simulink model "GP_DataCollection_2R"  (R2024a)
settings: Solver=ode4  StartTime=0.0  StopTime=6  FixedStep=0.001  RelTol=1e-3
model workspace (MAT data in the model file):
  p_hat.a1 = 1
  p_hat.a2 = 1
  p_hat.m1 = 2
  p_hat.m2 = 1
  p_hat.mm1 = 0.5
  p_hat.mm2 = 0.3
  p_hat.l1 = 0.5
  p_hat.l2 = 0.5
  p_hat.I1 = 0.166666666667
  p_hat.I2 = 0.0833333333333
  p_hat.kr1 = 50
  p_hat.kr2 = 50
  p_hat.Im1 = 0.0001
  p_hat.Im2 = 0.0001
  p_hat.g0 = 9.81
  p_real.a1 = 1
  p_real.a2 = 1
  p_real.m1 = 2
  p_real.m2 = 1
  p_real.mm1 = 0.5
  p_real.mm2 = 0.3
  p_real.l1 = 0.5
  p_real.l2 = 0.5
  p_real.I1 = 0.166666666667
  p_real.I2 = 0.0833333333333
  p_real.kr1 = 50
  p_real.kr2 = 50
  p_real.Im1 = 0.0001
  p_real.Im2 = 0.0001
  p_real.g0 = 9.81
undefined symbols (not defined in the file): dq0, Kd, Kp, q0
settings Model: Creator=Mariapaola  LastModifiedBy=Mariapaola

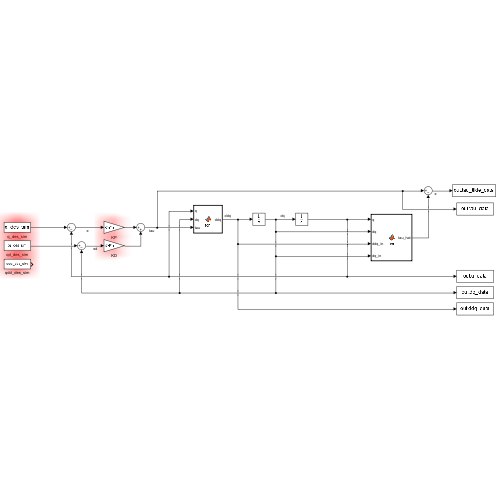
[thumbnail: Simulink's stored preview of the top-level diagram]
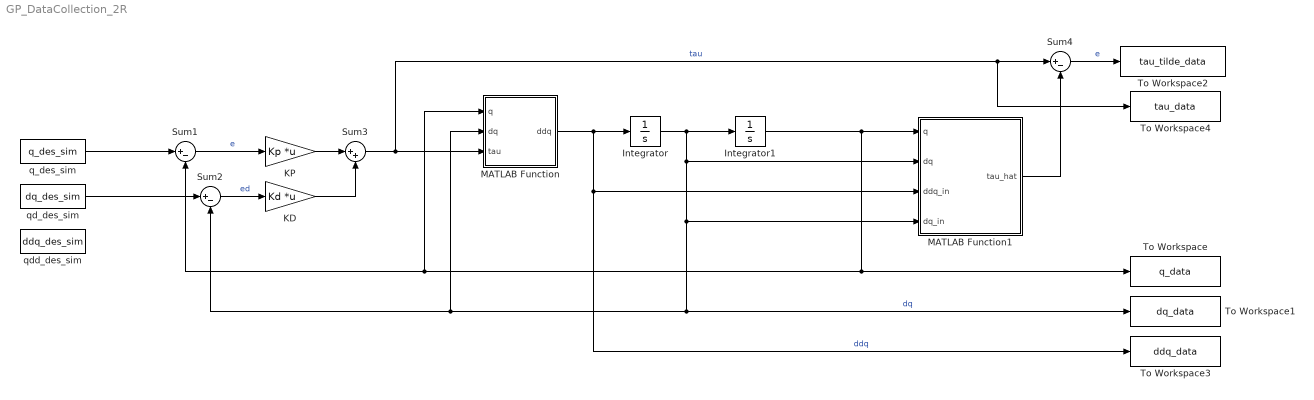
== system GP_DataCollection_2R ==
  Integrator : Integrator  InitialCondition=dq0
  Integrator1 : Integrator  InitialCondition=q0
  KD : Gain  Gain=Kd  Multiplication=Matrix(K*u)
  KP : Gain  Gain=Kp  Multiplication=Matrix(K*u)
  MATLAB Function : MATLAB Function  TreatAsAtomicUnit=on
  MATLAB Function1 : MATLAB Function  TreatAsAtomicUnit=on
  Sum1 : Sum  Inputs=|+-
  Sum2 : Sum  Inputs=|+-
  Sum3 : Sum  Inputs=|++
  Sum4 : Sum  Inputs=|+-
  To Workspace : ToWorkspace  VariableName=q_data  SampleTime=-1
  To Workspace1 : ToWorkspace  VariableName=dq_data  SampleTime=-1
  To Workspace2 : ToWorkspace  VariableName=tau_tilde_data  SaveFormat=Timeseries  SampleTime=-1
  To Workspace3 : ToWorkspace  VariableName=ddq_data  SampleTime=-1
  To Workspace4 : ToWorkspace  VariableName=tau_data  SaveFormat=Timeseries  SampleTime=-1
  "q_des_sim " : FromWorkspace  VariableName=q_des_sim
  qd_des_sim : FromWorkspace  VariableName=dq_des_sim
  qdd_des_sim : FromWorkspace  VariableName=ddq_des_sim
  wires:
  Integrator/1 -> Integrator1/1, MATLAB Function1/2(dq), MATLAB Function1/4(dq_in), To Workspace1/1, MATLAB Function/2(dq), Sum2/2  "dq"
  Sum2/1 -> KD/1  "ed"
  Sum1/1 -> KP/1  "e"
  KP/1 -> Sum3/1
  KD/1 -> Sum3/2
  Sum3/1 -> MATLAB Function/3(tau), Sum4/1, To Workspace4/1  "tau"
  "q_des_sim "/1 -> Sum1/1
  qd_des_sim/1 -> Sum2/1
  MATLAB Function/1(ddq) -> Integrator/1, MATLAB Function1/3(ddq_in), To Workspace3/1  "ddq"
  MATLAB Function1/1(tau_hat) -> Sum4/2
  Sum4/1 -> To Workspace2/1  "e"
  Integrator1/1 -> MATLAB Function/1(q), Sum1/2, To Workspace/1, MATLAB Function1/1(q)

== matlab function GP_DataCollection_2R/MATLAB Function1 ==
  data: q input; tau_hat output; dq input; ddq_in input; dq_in input
function tau_hat  = fcn(q,dq,ddq_in,dq_in)

tau_hat = computed_torque_model(q,dq,ddq_in,dq_in);

end

== matlab function GP_DataCollection_2R/MATLAB Function ==
  data: q input; ddq output; dq input; tau input
function ddq = fcn(q,dq,tau)

ddq = dynamics_model(q,dq,tau);

end
